simulink library "wing_downwash_lib"  (R2018b)
settings: Solver=VariableStepAuto  StartTime=0.0  StopTime=10.0  RelTol=1e-3
undefined symbols (not defined in the file or in its folder): downwash
libraries: $bdroot x1, linear_systems_lib x1, simulink x1
settings Model: Creator=Ybeyer  LastModifiedBy=yannic
settings SFSimCC: SimUseLocalCustomCode=off
settings RTWCC: RTWUseLocalCustomCode=off
settings CodeAppCC: StateflowObjectComments=on

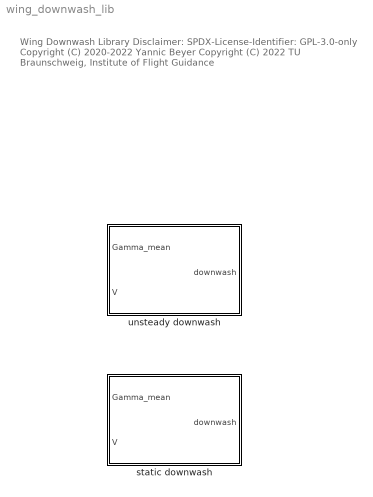
== system wing_downwash_lib ==
  note: Wing Downwash Library
      |
      | Disclaimer:
      | SPDX-License-Identifier: GPL-3.0-only
      |
      | Copyright (C) 2020-2022 Yannic Beyer
      | Copyright (C) 2022 TU Braunschweig, Institute of Flight Guidance
  static downwash : Subsystem  mask{downwash=downwash}
      mask prompts: downwash "downwash struct (see aircraftDownwash)"
      mask DialogControl DescGroupVar Prompt: Static downwash
      mask DialogControl DescTextVar Prompt: Transport delay depending on airspeed for modeling downwash of front wing to aft wing
      mask DialogControl Control2 Prompt: Inputs:
      mask DialogControl Control3 Prompt: Gamma_mean: mean circulation of front wing
      mask DialogControl Control4 Prompt: V: airspeed
      mask DialogControl Control5 Prompt: Outputs:
      mask DialogControl Control6 Prompt: vertical induced velocity (w)
  unsteady downwash : Subsystem  mask{downwash=downwash}
      mask prompts: downwash "downwash struct (see downwashUnstFromVlmWings)"
      mask init:
      | % create bus object downwash_bus in base workspace
      | struct2bus(downwash);
      mask DialogControl DescGroupVar Prompt: Unsteady downwash
      mask DialogControl DescTextVar Prompt: Transport delay and transfer function depending on airspeed for modeling downwash of front wing to aft wing
      mask DialogControl Control2 Prompt: Inputs:
      mask DialogControl Control3 Prompt: Gamma_mean: mean circulation of front wing
      mask DialogControl Control4 Prompt: V: airspeed
      mask DialogControl Control5 Prompt: Outputs:
      mask DialogControl Control6 Prompt: vertical induced velocity (w) and its derivative (w_dt)

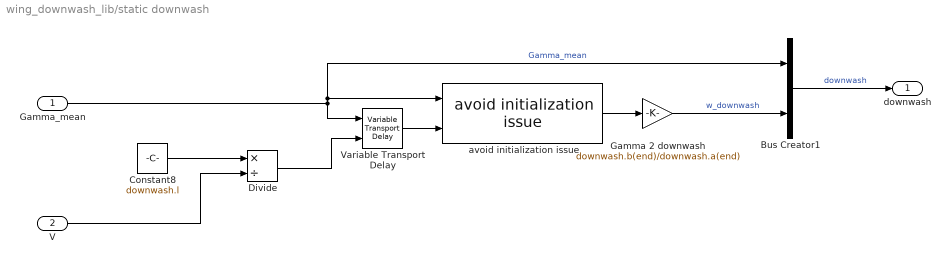
== system wing_downwash_lib/static downwash ==
  Gamma_mean : Inport
  V : Inport  Port=2
  Bus Creator1 : BusCreator  Inputs=2
  Constant8 : Constant  Value=downwash.l  OutDataTypeStr=Inherit: Inherit via back propagation
  Divide : Product  Inputs=*/
  Gamma 2 downwash : Gain  Gain=downwash.b(end)/downwash.a(end)
  Variable Transport Delay : VariableTransportDelay  VariableDelayType=Variable transport delay  MaximumDelay=10
  avoid initialization issue : $bdroot/unsteady downwash/avoid initialization issue  SystemSampleTime=-1
  downwash : Outport
  wires:
  Constant8/1 -> Divide/1
  Gamma 2 downwash/1 -> Bus Creator1/2  "w_downwash"
  Gamma_mean/1 -> Variable Transport Delay/1, avoid initialization issue/1, Bus Creator1/1  "Gamma_mean"
  Divide/1 -> Variable Transport Delay/2
  Variable Transport Delay/1 -> avoid initialization issue/2
  V/1 -> Divide/2
  Bus Creator1/1 -> downwash/1  "downwash"
  avoid initialization issue/1 -> Gamma 2 downwash/1

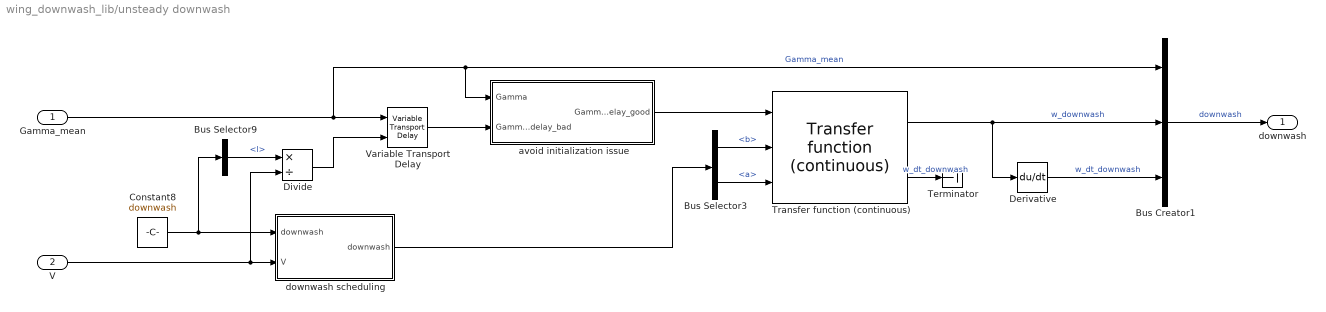
== system wing_downwash_lib/unsteady downwash ==
  Gamma_mean : Inport
  V : Inport  Port=2
  Bus Creator1 : BusCreator  Inputs=3
  Bus Selector3 : BusSelector  OutputSignals=b,a
  Bus Selector9 : BusSelector  OutputSignals=l
  Constant8 : Constant  Value=downwash  OutDataTypeStr=Bus: downwash_bus
  Derivative : Derivative
  Divide : Product  Inputs=*/
  Terminator : Terminator
  Transfer function (continuous) : linear_systems_lib/Transfer function (continuous)
      settings: SourceProductName=LADAC
  Variable Transport Delay : VariableTransportDelay  VariableDelayType=Variable transport delay  MaximumDelay=10
  avoid initialization issue : Subsystem
  downwash scheduling : MATLAB Function  TreatAsAtomicUnit=on
  downwash : Outport
  wires:
  Bus Selector9/1 -> Divide/1  "<l>"
  Transfer function (continuous)/1 -> Derivative/1, Bus Creator1/2  "w_downwash"
  Gamma_mean/1 -> Bus Creator1/1, avoid initialization issue/1(Gamma), Variable Transport Delay/1  "Gamma_mean"
  Divide/1 -> Variable Transport Delay/2
  Transfer function (continuous)/2 -> Terminator/1  "w_dt_downwash"
  downwash scheduling/1(downwash) -> Bus Selector3/1
  Constant8/1 -> downwash scheduling/1("downwash "), Bus Selector9/1
  Derivative/1 -> Bus Creator1/3  "w_dt_downwash"
  V/1 -> downwash scheduling/2(V), Divide/2
  Bus Selector3/2 -> Transfer function (continuous)/3  "<a>"
  Bus Selector3/1 -> Transfer function (continuous)/2  "<b>"
  Bus Creator1/1 -> downwash/1  "downwash"
  Variable Transport Delay/1 -> avoid initialization issue/2(Gamma_delay_bad)
  avoid initialization issue/1(Gamma_delay_good) -> Transfer function (continuous)/1

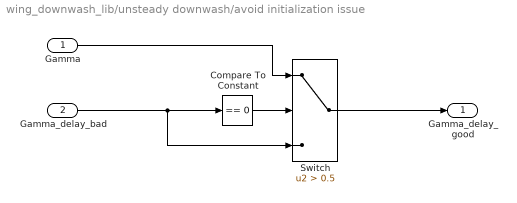
== system wing_downwash_lib/unsteady downwash/avoid initialization issue ==
  Gamma : Inport
  Gamma_delay_bad : Inport  Port=2
  Compare To Constant : simulink/Logic and Bit Operations/Compare To Constant  relop===  const=0  OutDataTypeStr=boolean
  Switch : Switch  Criteria=u2 > Threshold  Threshold=0.5
  Gamma_delay_good : Outport
  wires:
  Compare To Constant/1 -> Switch/2
  Gamma_delay_bad/1 -> Switch/3, Compare To Constant/1
  Switch/1 -> Gamma_delay_good/1
  Gamma/1 -> Switch/1

== matlab function wing_downwash_lib/unsteady downwash/downwash scheduling ==
  data: downwash input Bus: downwash_bus; downwash output; V input
function downwash = fcn(downwash, V)
downwash = downwashUnstSchedule(downwash,V);
end
